simulink model "HW1_7_feedforward_no"  (R2025b)
settings: Solver=VariableStepAuto  StartTime=0.0  StopTime=10.0  RelTol=1e-3
settings Model: Creator=bcc  LastModifiedBy=bcc

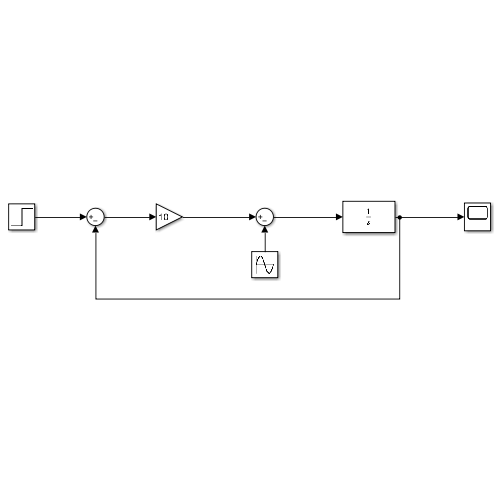
[thumbnail: Simulink's stored preview of the top-level diagram]
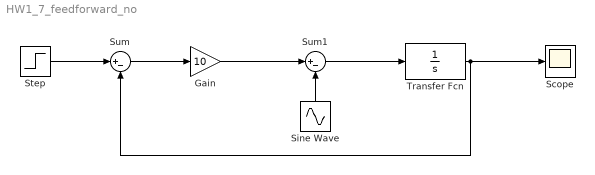
== system HW1_7_feedforward_no ==
  Gain : Gain  Gain=10
  Scope : Scope
      settings: ActiveDisplayYMinimum=-0.52852862358414066  ActiveDisplayYMaximum=1.5157822002727479
  Sine Wave : Sin  Amplitude=5  Frequency=4*pi  SampleTime=0
  Step : Step  SampleTime=0
  Sum : Sum  Inputs=|+-
  Sum1 : Sum  Inputs=|+-
  Transfer Fcn : TransferFcn  Denominator=[1 0]
  wires:
  Step/1 -> Sum/1
  Sum/1 -> Gain/1
  Transfer Fcn/1 -> Sum/2, Scope/1
  Gain/1 -> Sum1/1
  Sum1/1 -> Transfer Fcn/1
  Sine Wave/1 -> Sum1/2
